simulink model "morilla_test_simu"  (R2024a)
settings: Solver=VariableStepAuto  StartTime=0.0  StopTime=300  RelTol=1e-3
values from neighbouring files (symbols this model uses):
  Dc = cell(2)    [morilla_exemplos.m]
  Gr = tf(Nc_g, Dc_g)    [morilla_exemplos.m]
  k_i = k    [morilla_exemplos.m]
  tau_pid = zeros(2)    [desacoplador_cCentralizado.m]    (also in morilla_exemplos.m = tauK)
  Tau_tot = totaldelay(G)    [desacoplador_cCentralizado.m]    (also in morilla_exemplos.m = theta)
libraries: slpidlib x2
settings Model: Creator=Déborah Silva  LastModifiedBy=Déborah Silva

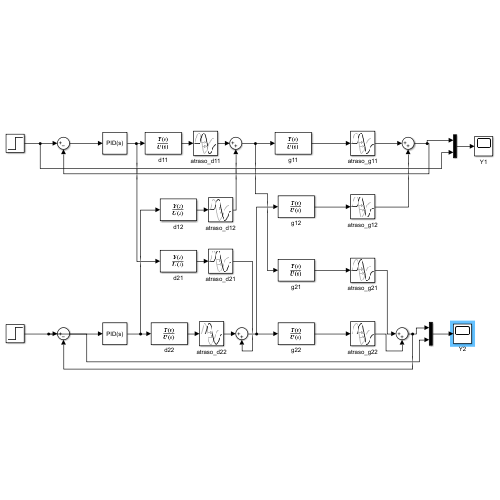
[thumbnail: Simulink's stored preview of the top-level diagram]
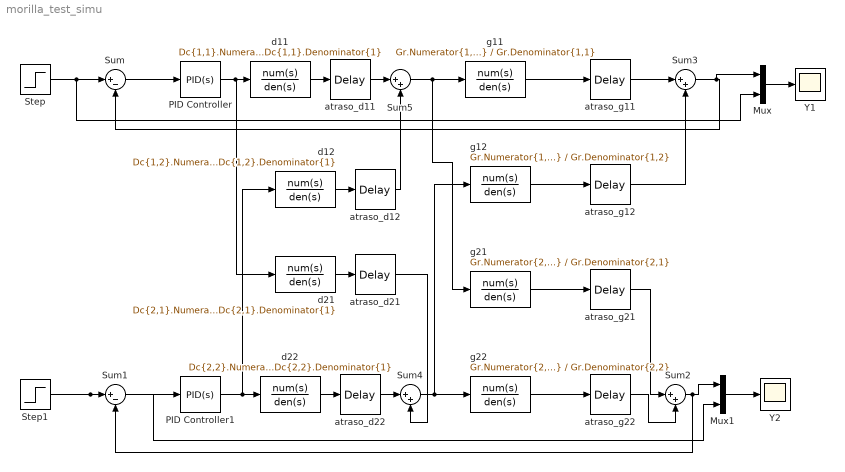
== system morilla_test_simu ==
  Mux : Mux  Inputs=2
  Mux1 : Mux  Inputs=2
  PID Controller : slpidlib/PID Controller  Controller=PID  Form=Parallel  TimeDomain=Continuous-time  UseExternalTs=off  SampleTime=-1  IntegratorMethod=Forward Euler  FilterMethod=Forward Euler  ControllerParametersSource=internal  P=k_i(1)  I=0  UseKiTs=off  D=0  UseExternalDerivativeSource=off  N=100  UseFilter=on  TunerSelectOption=Transfer Function Based (PID Tuner App)  InitialConditionSource=internal  InitialConditionForIntegrator=0  InitialConditionForFilter=0  DifferentiatorICPrevScaledInput=0  ExternalReset=none  TrackingMode=off  Kt=1  LimitOutput=off  SatLimitsSource=internal  UpperSaturationLimit=inf  LowerSaturationLimit=-inf  LinearizeAsGain=on  AntiWindupMode=none  Kb=1  LimitIntegrator=off  UpperIntegratorSaturationLimit=inf  LowerIntegratorSaturationLimit=-inf  POutMin=[]  POutMax=[]  IOutMin=[]  IOutMax=[]  DOutMin=[]  DOutMax=[]  NOutMin=[]  NOutMax=[]  SumOutMin=[]  SumOutMax=[]  SaturationOutMin=[]  SaturationOutMax=[]  PParamMin=[]  PParamMax=[]  IParamMin=[]  IParamMax=[]  DParamMin=[]  DParamMax=[]  NParamMin=[]  NParamMax=[]  KbParamMin=[]  KbParamMax=[]  KtParamMin=[]  KtParamMax=[]  KbOutMin=[]  KbOutMax=[]  KtOutMin=[]  KtOutMax=[]  IntegratorOutMin=[]  IntegratorOutMax=[]  FilterOutMin=[]  FilterOutMax=[]  SumI1OutMin=[]  SumI1OutMax=[]  SumI2OutMin=[]  SumI2OutMax=[]  SumI3OutMin=[]  SumI3OutMax=[]  SumI4OutMin=[]  SumI4OutMax=[]  SumDOutMin=[]  SumDOutMax=[]  DifferentiatorOutMin=[]  DifferentiatorOutMax=[]  FilterDiffOutCoefMin=[]  FilterDiffOutCoefMax=[]  ReciprocalOutMin=[]  ReciprocalOutMax=[]  SumDenOutMin=[]  SumDenOutMax=[]  SumNumOutMin=[]  SumNumOutMax=[]  DivideOutMin=[]  DivideOutMax=[]  UdiffTsProdOutMin=[]  UdiffTsProdOutMax=[]  NTsProdOutMin=[]  NTsProdOutMax=[]  UintegralTsProdOutMin=[]  UintegralTsProdOutMax=[]  UngainTsProdOutMin=[]  UngainTsProdOutMax=[]  ClampingZeroOutDataTypeStr=Inherit: Inherit via back propagation  ClampingZeroOutMin=[]  ClampingZeroOutMax=[]  FilterDenConstantOutDataTypeStr=Inherit: Inherit via back propagation  FilterDenConstantOutMin=[]  FilterDenConstantOutMax=[]  PCopyOutDataTypeStr=Inherit: Inherit via back propagation  PCopyOutMin=[]  PCopyOutMax=[]  NCopyOutDataTypeStr=Inherit: Inherit via back propagation  NCopyOutMin=[]  NCopyOutMax=[]  IntegratorContinuousStateAttributes=''  IntegratorStateMustResolveToSignalObject=off  IntegratorRTWStateStorageClass=Auto  FilterContinuousStateAttributes=''  FilterStateMustResolveToSignalObject=off  FilterRTWStateStorageClass=Auto  ParallelPVariant=InternalParameters  IdealPVariant=Disabled  IVariant=InternalParameters  DVariant=InternalParameters  IntegratorVariant=Continuous  SatVariant=Disabled  AWVariant=Passthrough  PCopyVariant=Disabled  TRVariant=Disabled  FdbkBlocksVariant=Forward  IdealPFdbkVariant=Disabled  SatFdbkVariant=Disabled  DerivativeFilterVariant=ContFilter  NVariant=InternalParameters  NCopyVariant=Disabled  FilterICVariant=InternalICsFilter  IntegratorICVariant=InternalICs  ExternalResetVariant=Disabled  TRSumVariant=Passthrough  SumFdbkVariant=Disabled  SumVariant=Sum_PID  TsampFilterVariant=InternalTs  TsampNgainVariant=Passthrough  TsampIntegralVariant=Disabled_SignalSpec  ExternalSaturationOutDataTypeStr=Inherit: Same as second input  DerivativeSourceVariant=ErrorSignal
  PID Controller1 : slpidlib/PID Controller  Controller=PID  Form=Parallel  TimeDomain=Continuous-time  UseExternalTs=off  SampleTime=-1  IntegratorMethod=Forward Euler  FilterMethod=Forward Euler  ControllerParametersSource=internal  P=k_i(2)  I=0  UseKiTs=off  D=0  UseExternalDerivativeSource=off  N=100  UseFilter=on  TunerSelectOption=Transfer Function Based (PID Tuner App)  InitialConditionSource=internal  InitialConditionForIntegrator=0  InitialConditionForFilter=0  DifferentiatorICPrevScaledInput=0  ExternalReset=none  TrackingMode=off  Kt=1  LimitOutput=off  SatLimitsSource=internal  UpperSaturationLimit=inf  LowerSaturationLimit=-inf  LinearizeAsGain=on  AntiWindupMode=none  Kb=1  LimitIntegrator=off  UpperIntegratorSaturationLimit=inf  LowerIntegratorSaturationLimit=-inf  POutMin=[]  POutMax=[]  IOutMin=[]  IOutMax=[]  DOutMin=[]  DOutMax=[]  NOutMin=[]  NOutMax=[]  SumOutMin=[]  SumOutMax=[]  SaturationOutMin=[]  SaturationOutMax=[]  PParamMin=[]  PParamMax=[]  IParamMin=[]  IParamMax=[]  DParamMin=[]  DParamMax=[]  NParamMin=[]  NParamMax=[]  KbParamMin=[]  KbParamMax=[]  KtParamMin=[]  KtParamMax=[]  KbOutMin=[]  KbOutMax=[]  KtOutMin=[]  KtOutMax=[]  IntegratorOutMin=[]  IntegratorOutMax=[]  FilterOutMin=[]  FilterOutMax=[]  SumI1OutMin=[]  SumI1OutMax=[]  SumI2OutMin=[]  SumI2OutMax=[]  SumI3OutMin=[]  SumI3OutMax=[]  SumI4OutMin=[]  SumI4OutMax=[]  SumDOutMin=[]  SumDOutMax=[]  DifferentiatorOutMin=[]  DifferentiatorOutMax=[]  FilterDiffOutCoefMin=[]  FilterDiffOutCoefMax=[]  ReciprocalOutMin=[]  ReciprocalOutMax=[]  SumDenOutMin=[]  SumDenOutMax=[]  SumNumOutMin=[]  SumNumOutMax=[]  DivideOutMin=[]  DivideOutMax=[]  UdiffTsProdOutMin=[]  UdiffTsProdOutMax=[]  NTsProdOutMin=[]  NTsProdOutMax=[]  UintegralTsProdOutMin=[]  UintegralTsProdOutMax=[]  UngainTsProdOutMin=[]  UngainTsProdOutMax=[]  ClampingZeroOutDataTypeStr=Inherit: Inherit via back propagation  ClampingZeroOutMin=[]  ClampingZeroOutMax=[]  FilterDenConstantOutDataTypeStr=Inherit: Inherit via back propagation  FilterDenConstantOutMin=[]  FilterDenConstantOutMax=[]  PCopyOutDataTypeStr=Inherit: Inherit via back propagation  PCopyOutMin=[]  PCopyOutMax=[]  NCopyOutDataTypeStr=Inherit: Inherit via back propagation  NCopyOutMin=[]  NCopyOutMax=[]  IntegratorContinuousStateAttributes=''  IntegratorStateMustResolveToSignalObject=off  IntegratorRTWStateStorageClass=Auto  FilterContinuousStateAttributes=''  FilterStateMustResolveToSignalObject=off  FilterRTWStateStorageClass=Auto  ParallelPVariant=InternalParameters  IdealPVariant=Disabled  IVariant=InternalParameters  DVariant=InternalParameters  IntegratorVariant=Continuous  SatVariant=Disabled  AWVariant=Passthrough  PCopyVariant=Disabled  TRVariant=Disabled  FdbkBlocksVariant=Forward  IdealPFdbkVariant=Disabled  SatFdbkVariant=Disabled  DerivativeFilterVariant=ContFilter  NVariant=InternalParameters  NCopyVariant=Disabled  FilterICVariant=InternalICsFilter  IntegratorICVariant=InternalICs  ExternalResetVariant=Disabled  TRSumVariant=Passthrough  SumFdbkVariant=Disabled  SumVariant=Sum_PID  TsampFilterVariant=InternalTs  TsampNgainVariant=Passthrough  TsampIntegralVariant=Disabled_SignalSpec  ExternalSaturationOutDataTypeStr=Inherit: Same as second input  DerivativeSourceVariant=ErrorSignal
  Step : Step  SampleTime=0
  Step1 : Step  Time=60  SampleTime=0
  Sum : Sum  Inputs=|+-
  Sum1 : Sum  Inputs=|+-
  Sum{2..5} (4 alike) : Sum  Inputs=|++
  Y1 : Scope
  Y2 : Scope
  atraso_d11 : TransportDelay  DelayTime=tau_pid(1,1)
  atraso_d12 : TransportDelay  DelayTime=tau_pid(1,2)
  atraso_d21 : TransportDelay  DelayTime=tau_pid(2,1)
  atraso_d22 : TransportDelay  DelayTime=tau_pid(2,2)
  atraso_g11 : TransportDelay  DelayTime=Tau_tot(1,1)
  atraso_g12 : TransportDelay  DelayTime=Tau_tot(1,2)
  atraso_g21 : TransportDelay  DelayTime=Tau_tot(2,1)
  atraso_g22 : TransportDelay  DelayTime=Tau_tot(2,2)
  d11 : TransferFcn  Numerator=Dc{1,1}.Numerator{1}  Denominator=Dc{1,1}.Denominator{1}
  d12 : TransferFcn  Numerator=Dc{1,2}.Numerator{1}  Denominator=Dc{1,2}.Denominator{1}
  d21 : TransferFcn  Numerator=Dc{2,1}.Numerator{1}  Denominator=Dc{2,1}.Denominator{1}
  d22 : TransferFcn  Numerator=Dc{2,2}.Numerator{1}  Denominator=Dc{2,2}.Denominator{1}
  g11 : TransferFcn  Numerator=Gr.Numerator{1,1}  Denominator=Gr.Denominator{1,1}
  g12 : TransferFcn  Numerator=Gr.Numerator{1,2}  Denominator=Gr.Denominator{1,2}
  g21 : TransferFcn  Numerator=Gr.Numerator{2,1}  Denominator=Gr.Denominator{2,1}
  g22 : TransferFcn  Numerator=Gr.Numerator{2,2}  Denominator=Gr.Denominator{2,2}
  wires:
  PID Controller/1 -> d21/1, d11/1
  Sum5/1 -> g21/1, g11/1
  Mux/1 -> Y1/1
  Mux1/1 -> Y2/1
  Sum2/1 -> Sum1/2, Mux1/1
  Sum3/1 -> Mux/1, Sum/2
  Step/1 -> Mux/2, Sum/1
  Sum/1 -> PID Controller/1
  PID Controller1/1 -> d12/1, d22/1
  Sum4/1 -> g12/1, g22/1
  Step1/1 -> Mux1/2, Sum1/1
  Sum1/1 -> PID Controller1/1
  g11/1 -> atraso_g11/1
  atraso_g11/1 -> Sum3/1
  atraso_g12/1 -> Sum3/2
  g12/1 -> atraso_g12/1
  g21/1 -> atraso_g21/1
  g22/1 -> atraso_g22/1
  atraso_g22/1 -> Sum2/2
  atraso_g21/1 -> Sum2/1
  d11/1 -> atraso_d11/1
  atraso_d11/1 -> Sum5/1
  d12/1 -> atraso_d12/1
  d21/1 -> atraso_d21/1
  d22/1 -> atraso_d22/1
  atraso_d22/1 -> Sum4/1
  atraso_d21/1 -> Sum4/2
  atraso_d12/1 -> Sum5/2
